simulink model "ASM_Traffic_MultiCore"  (R2026a)
settings: Solver=ode1  StartTime=SIM.tstart.v  StopTime=SIM.tend.v  FixedStep=SIM.StepSize.v
PostLoadFcn:
  | if any(exist('dsrtsu_mdlpostloadfcn', 'file') ~= 0), dsrtsu_mdlpostloadfcn('Execute', bdroot); end
  | try, asm_mdl_postloadfcn(bdroot, 'UpdateModel', 3600); catch, disp(lasterr); end,
InitFcn:
  | , if any(exist('rtifpga_mdlclblib', 'file') ~= 0), rtifpga_mdlclblib('Init', bdroot); end,
  | , if any(exist('dsmpb_private', 'file') ~= 0), dsmpb_private('dsmpb_mdlclblib', 'Init', bdroot); end,
model workspace (MAT data in the model file):
  asmReferencePath = [0 0.01 0.02 0.03 0.04 0.05 0.06 0.07 0.08 0.09 0.1 0.11 ... (350007 elements, 50001x7)]
  roadBounds : Simulink.Parameter (value not decoded)
  safetyAxes : Simulink.Parameter (value not decoded)
undefined symbols (not defined in the file): _to_, a0b2, ASM_BrakeHydraulics_DemoSystems, ASM_VehicleDynamics_DemoSystems, b98103fe8ad365046cd0, BrakeCircuit, controllerConfig, CPT, Crankshaft, DiscIntNeverNeededParam, dsmsi, FinalDriveAssembly, MDL, ModeSignals, mu, Pos_BrakePedal_Maneuver, rad, RefSignals, roadFamilyData, roadFamilyId, s_to_rpm, SIM, SoftECU, Suspension, Tire, Transmission
libraries: ASM_Traffic_lib x135, simulink x98, ASM_Utils_lib x77, ASM_VehicleDynamics_lib x70, ASM_Environment_lib x22, dsmpblib x20, dsmsilib x15, MDLD_Utils_lib x10, ASM_BrakeHydraulics_lib x3, sl_discontinuities x2
(part 43 of 65)

== system ASM_Traffic_MultiCore/Environment/Traffic/PlantModel/FellowMovement/Customize_UserSignals ==
  UserSignals_In : Inport
  UserSignalsFellow_In : Inport  Port=2
  Bus Creator : BusCreator  Inputs=3
  Bus Creator1 : BusCreator  Inputs=213
  Bus Selector : BusSelector  OutputSignals=User1[]
  Bus Selector1 : BusSelector  OutputSignals=User2[],User3[],User4[]
  Bus Selector2 : BusSelector  OutputSignals=User1[],User2[],User3[],User4[],User5[],User6[],User7[],User8[],User9[],User10[]
  Demux{,1..6} (7 alike) : Demux  Outputs=MDL.Traffic.MaxNumFellows.v
  Gain : Gain
  Gain1 : Gain
  Gain2 : Gain
  Memory : UnitDelay  SampleTime=-1
  Mux : Mux  Inputs=10
  Saturation : Saturate  UpperLimit=1  LowerLimit=0
  Select_1 : Selector  InputPortWidth=MDL.Traffic.MaxNumFellows.v*MDL.Traffic.MaxNumFDUserSignals.v  IndexOptions=Index vector (dialog)  Indices=[1:MDL.Traffic.MaxNumFDUserSignals.v:MDL.Traffic.MaxNumFellows.v*MDL.Traffic.MaxNumFDUserSignals.v]  OutputSizes=1
  Select_2 : Selector  InputPortWidth=MDL.Traffic.MaxNumFellows.v*MDL.Traffic.MaxNumFDUserSignals.v  IndexOptions=Index vector (dialog)  Indices=[2:MDL.Traffic.MaxNumFDUserSignals.v:MDL.Traffic.MaxNumFellows.v*MDL.Traffic.MaxNumFDUserSignals.v]  OutputSizes=1
  Select_3 : Selector  InputPortWidth=MDL.Traffic.MaxNumFellows.v*MDL.Traffic.MaxNumFDUserSignals.v  IndexOptions=Index vector (dialog)  Indices=[3:MDL.Traffic.MaxNumFDUserSignals.v:MDL.Traffic.MaxNumFellows.v*MDL.Traffic.MaxNumFDUserSignals.v]  OutputSizes=1
  Select_4 : Selector  InputPortWidth=MDL.Traffic.MaxNumFellows.v*MDL.Traffic.MaxNumFDUserSignals.v  IndexOptions=Index vector (dialog)  Indices=[4:MDL.Traffic.MaxNumFDUserSignals.v:MDL.Traffic.MaxNumFellows.v*MDL.Traffic.MaxNumFDUserSignals.v]  OutputSizes=1
  Select_5 : Selector  InputPortWidth=MDL.Traffic.MaxNumFellows.v*MDL.Traffic.MaxNumFDUserSignals.v  IndexOptions=Index vector (dialog)  Indices=[5:MDL.Traffic.MaxNumFDUserSignals.v:MDL.Traffic.MaxNumFellows.v*MDL.Traffic.MaxNumFDUserSignals.v]  OutputSizes=1
  Select_6 : Selector  InputPortWidth=MDL.Traffic.MaxNumFellows.v*MDL.Traffic.MaxNumFDUserSignals.v  IndexOptions=Index vector (dialog)  Indices=[6:MDL.Traffic.MaxNumFDUserSignals.v:MDL.Traffic.MaxNumFellows.v*MDL.Traffic.MaxNumFDUserSignals.v]  OutputSizes=1
  Select_7 : Selector  InputPortWidth=MDL.Traffic.MaxNumFellows.v*MDL.Traffic.MaxNumFDUserSignals.v  IndexOptions=Index vector (dialog)  Indices=[7:MDL.Traffic.MaxNumFDUserSignals.v:MDL.Traffic.MaxNumFellows.v*MDL.Traffic.MaxNumFDUserSignals.v]  OutputSizes=1
  Select_8 : Selector  InputPortWidth=MDL.Traffic.MaxNumFellows.v*MDL.Traffic.MaxNumFDUserSignals.v  IndexOptions=Index vector (dialog)  Indices=[8:MDL.Traffic.MaxNumFDUserSignals.v:MDL.Traffic.MaxNumFellows.v*MDL.Traffic.MaxNumFDUserSignals.v]  OutputSizes=1
  Sum : Sum  Inputs=|-+  SaturateOnIntegerOverflow=on
  ASMSignalBus : Outport  VectorParamsAs1DForOutWhenUnconnected=off
  Movement_Characteristics[] : Outport  Port=2  VectorParamsAs1DForOutWhenUnconnected=off
  wires:
  Select_2/1 -> Movement_Characteristics[]/1
  Select_1/1 -> Demux/1
  UserSignalsFellow_In/1 -> Select_1/1, Select_2/1, Select_3/1, Select_8/1, Select_7/1, Select_6/1, Select_5/1, Select_4/1
  UserSignals_In/1 -> Bus Selector2/1, Bus Selector1/1, Bus Selector/1  "UserSignals"
  Bus Selector/1 -> Sum/2, Memory/1  "<User1[]>"
  Saturation/1 -> Bus Creator1/1  "ManeuverSegmentEndTrigger[0|1]"
  Bus Creator1/1 -> ASMSignalBus/1  "UserSignals_Customized"
  Sum/1 -> Saturation/1
  Memory/1 -> Sum/1
  Demux/1 -> Bus Creator1/4  "Fellow1_TurnLights"
  Demux/30 -> Bus Creator1/33  "Fellow30_TurnLights"
  Demux/2 -> Bus Creator1/5  "Fellow2_TurnLights"
  Demux/3 -> Bus Creator1/6  "Fellow3_TurnLights"
  Demux/4 -> Bus Creator1/7  "Fellow4_TurnLights"
  Demux/5 -> Bus Creator1/8  "Fellow5_TurnLights"
  Demux/6 -> Bus Creator1/9  "Fellow6_TurnLights"
  Demux/7 -> Bus Creator1/10  "Fellow7_TurnLights"
  Demux/8 -> Bus Creator1/11  "Fellow8_TurnLights"
  Demux/9 -> Bus Creator1/12  "Fellow9_TurnLights"
  Demux/10 -> Bus Creator1/13  "Fellow10_TurnLights"
  Demux/11 -> Bus Creator1/14  "Fellow11_TurnLights"
  Demux/12 -> Bus Creator1/15  "Fellow12_TurnLights"
  Demux/13 -> Bus Creator1/16  "Fellow13_TurnLights"
  Demux/14 -> Bus Creator1/17  "Fellow14_TurnLights"
  Demux/15 -> Bus Creator1/18  "Fellow15_TurnLights"
  Demux/16 -> Bus Creator1/19  "Fellow16_TurnLights"
  Demux/17 -> Bus Creator1/20  "Fellow17_TurnLights"
  Demux/18 -> Bus Creator1/21  "Fellow18_TurnLights"
  Demux/19 -> Bus Creator1/22  "Fellow19_TurnLights"
  Demux/20 -> Bus Creator1/23  "Fellow20_TurnLights"
  Demux/21 -> Bus Creator1/24  "Fellow21_TurnLights"
  Demux/22 -> Bus Creator1/25  "Fellow22_TurnLights"
  Demux/23 -> Bus Creator1/26  "Fellow23_TurnLights"
  Demux/24 -> Bus Creator1/27  "Fellow24_TurnLights"
  Demux/25 -> Bus Creator1/28  "Fellow25_TurnLights"
  Demux/26 -> Bus Creator1/29  "Fellow26_TurnLights"
  Demux/27 -> Bus Creator1/30  "Fellow27_TurnLights"
  Demux/28 -> Bus Creator1/31  "Fellow28_TurnLights"
  Demux/29 -> Bus Creator1/32  "Fellow29_TurnLights"
  Bus Selector2/1 -> Mux/1  "<User1[]>"
  Bus Selector2/2 -> Mux/2  "<User2[]>"
  Bus Selector2/3 -> Mux/3  "<User3[]>"
  Bus Selector2/4 -> Mux/4  "<User4[]>"
  Bus Selector2/5 -> Mux/5  "<User5[]>"
  Mux/1 -> Bus Creator1/3  "UserSignals"
  Demux1/30 -> Bus Creator1/63  "Fellow30_DoorFL"
  Demux1/27 -> Bus Creator1/60  "Fellow27_DoorFL"
  Demux1/25 -> Bus Creator1/58  "Fellow25_DoorFL"
  Demux1/28 -> Bus Creator1/61  "Fellow28_DoorFL"
  Demux1/24 -> Bus Creator1/57  "Fellow24_DoorFL"
  Demux1/29 -> Bus Creator1/62  "Fellow29_DoorFL"
  Demux1/22 -> Bus Creator1/55  "Fellow22_DoorFL"
  Demux1/20 -> Bus Creator1/53  "Fellow20_DoorFL"
  Demux1/21 -> Bus Creator1/54  "Fellow21_DoorFL"
  Demux1/23 -> Bus Creator1/56  "Fellow23_DoorFL"
  Demux1/19 -> Bus Creator1/52  "Fellow19_DoorFL"
  Demux1/18 -> Bus Creator1/51  "Fellow18_DoorFL"
  Demux1/16 -> Bus Creator1/49  "Fellow16_DoorFL"
  Demux1/15 -> Bus Creator1/48  "Fellow15_DoorFL"
  Demux1/12 -> Bus Creator1/45  "Fellow12_DoorFL"
  Demux1/17 -> Bus Creator1/50  "Fellow17_DoorFL"
  Demux1/11 -> Bus Creator1/44  "Fellow11_DoorFL"
  Demux1/9 -> Bus Creator1/42  "Fellow9_DoorFL"
  Demux1/10 -> Bus Creator1/43  "Fellow10_DoorFL"
  Demux1/13 -> Bus Creator1/46  "Fellow13_DoorFL"
  Demux1/3 -> Bus Creator1/36  "Fellow3_DoorFL"
  Select_3/1 -> Demux1/1
  Demux1/7 -> Bus Creator1/40  "Fellow7_DoorFL"
  Demux1/8 -> Bus Creator1/41  "Fellow8_DoorFL"
  Demux1/26 -> Bus Creator1/59  "Fellow26_DoorFL"
  Demux1/6 -> Bus Creator1/39  "Fellow6_DoorFL"
  Demux1/14 -> Bus Creator1/47  "Fellow14_DoorFL"
  Demux1/2 -> Bus Creator1/35  "Fellow2_DoorFL"
  Demux1/5 -> Bus Creator1/38  "Fellow5_DoorFL"
  Demux1/4 -> Bus Creator1/37  "Fellow4_DoorFL"
  Demux1/1 -> Bus Creator1/34  "Fellow1_DoorFL"
  Demux2/30 -> Bus Creator1/93  "Fellow30_DoorFR"
  Demux2/27 -> Bus Creator1/90  "Fellow27_DoorFR"
  Demux2/25 -> Bus Creator1/88  "Fellow25_DoorFR"
  Demux2/28 -> Bus Creator1/91  "Fellow28_DoorFR"
  Demux2/24 -> Bus Creator1/87  "Fellow24_DoorFR"
  Demux2/29 -> Bus Creator1/92  "Fellow29_DoorFR"
  Demux2/22 -> Bus Creator1/85  "Fellow22_DoorFR"
  Demux2/20 -> Bus Creator1/83  "Fellow20_DoorFR"
  Demux2/21 -> Bus Creator1/84  "Fellow21_DoorFR"
  Demux2/23 -> Bus Creator1/86  "Fellow23_DoorFR"
  Demux2/19 -> Bus Creator1/82  "Fellow19_DoorFR"
  Demux2/18 -> Bus Creator1/81  "Fellow18_DoorFR"
  Demux2/16 -> Bus Creator1/79  "Fellow16_DoorFR"
  Demux2/15 -> Bus Creator1/78  "Fellow15_DoorFR"
  Demux2/12 -> Bus Creator1/75  "Fellow12_DoorFR"
  Demux2/17 -> Bus Creator1/80  "Fellow17_DoorFR"
  Demux2/11 -> Bus Creator1/74  "Fellow11_DoorFR"
  Demux2/9 -> Bus Creator1/72  "Fellow9_DoorFR"
  Demux2/10 -> Bus Creator1/73  "Fellow10_DoorFR"
  Demux2/13 -> Bus Creator1/76  "Fellow13_DoorFR"
  Demux2/3 -> Bus Creator1/66  "Fellow3_DoorFR"
  Select_4/1 -> Demux2/1
  Demux2/7 -> Bus Creator1/70  "Fellow7_DoorFR"
  Demux2/8 -> Bus Creator1/71  "Fellow8_DoorFR"
  Demux2/26 -> Bus Creator1/89  "Fellow26_DoorFR"
  Demux2/6 -> Bus Creator1/69  "Fellow6_DoorFR"
  Demux2/14 -> Bus Creator1/77  "Fellow14_DoorFR"
  Demux2/2 -> Bus Creator1/65  "Fellow2_DoorFR"
  Demux2/5 -> Bus Creator1/68  "Fellow5_DoorFR"
  Demux2/4 -> Bus Creator1/67  "Fellow4_DoorFR"
  Demux2/1 -> Bus Creator1/64  "Fellow1_DoorFR"
  Demux3/30 -> Bus Creator1/123  "Fellow30_DoorRL"
  Demux3/27 -> Bus Creator1/120  "Fellow27_DoorRL"
  Demux3/25 -> Bus Creator1/118  "Fellow25_DoorRL"
  Demux3/28 -> Bus Creator1/121  "Fellow28_DoorRL"
  Demux3/24 -> Bus Creator1/117  "Fellow24_DoorRL"
  Demux3/29 -> Bus Creator1/122  "Fellow29_DoorRL"
  Demux3/22 -> Bus Creator1/115  "Fellow22_DoorRL"
  Demux3/20 -> Bus Creator1/113  "Fellow20_DoorRL"
  Demux3/21 -> Bus Creator1/114  "Fellow21_DoorRL"
  Demux3/23 -> Bus Creator1/116  "Fellow23_DoorRL"
  Demux3/19 -> Bus Creator1/112  "Fellow19_DoorRL"
  Demux3/18 -> Bus Creator1/111  "Fellow18_DoorRL"
  Demux3/16 -> Bus Creator1/109  "Fellow16_DoorRL"
  Demux3/15 -> Bus Creator1/108  "Fellow15_DoorRL"
  Demux3/12 -> Bus Creator1/105  "Fellow12_DoorRL"
  Demux3/17 -> Bus Creator1/110  "Fellow17_DoorRL"
  Demux3/11 -> Bus Creator1/104  "Fellow11_DoorRL"
  Demux3/9 -> Bus Creator1/102  "Fellow9_DoorRL"
  Demux3/10 -> Bus Creator1/103  "Fellow10_DoorRL"
  Demux3/13 -> Bus Creator1/106  "Fellow13_DoorRL"
  Demux3/3 -> Bus Creator1/96  "Fellow3_DoorRL"
  Select_5/1 -> Demux3/1
  Demux3/7 -> Bus Creator1/100  "Fellow7_DoorRL"
  Demux3/8 -> Bus Creator1/101  "Fellow8_DoorRL"
  Demux3/26 -> Bus Creator1/119  "Fellow26_DoorRL"
  Demux3/6 -> Bus Creator1/99  "Fellow6_DoorRL"
  Demux3/14 -> Bus Creator1/107  "Fellow14_DoorRL"
  Demux3/2 -> Bus Creator1/95  "Fellow2_DoorRL"
  Demux3/5 -> Bus Creator1/98  "Fellow5_DoorRL"
  Demux3/4 -> Bus Creator1/97  "Fellow4_DoorRL"
  Demux3/1 -> Bus Creator1/94  "Fellow1_DoorRL"
  Demux4/30 -> Bus Creator1/153  "Fellow30_DoorRR"
  Demux4/27 -> Bus Creator1/150  "Fellow27_DoorRR"
  Demux4/25 -> Bus Creator1/148  "Fellow25_DoorRR"
  Demux4/28 -> Bus Creator1/151  "Fellow28_DoorRR"
  Demux4/24 -> Bus Creator1/147  "Fellow24_DoorRR"
  Demux4/29 -> Bus Creator1/152  "Fellow29_DoorRR"
  Demux4/22 -> Bus Creator1/145  "Fellow22_DoorRR"
  Demux4/20 -> Bus Creator1/143  "Fellow20_DoorRR"
  Demux4/21 -> Bus Creator1/144  "Fellow21_DoorRR"
  Demux4/23 -> Bus Creator1/146  "Fellow23_DoorRR"
  Demux4/19 -> Bus Creator1/142  "Fellow19_DoorRR"
  Demux4/18 -> Bus Creator1/141  "Fellow18_DoorRR"
  Demux4/16 -> Bus Creator1/139  "Fellow16_DoorRR"
  Demux4/15 -> Bus Creator1/138  "Fellow15_DoorRR"
  Demux4/12 -> Bus Creator1/135  "Fellow12_DoorRR"
  Demux4/17 -> Bus Creator1/140  "Fellow17_DoorRR"
  Demux4/11 -> Bus Creator1/134  "Fellow11_DoorRR"
  Demux4/9 -> Bus Creator1/132  "Fellow9_DoorRR"
  Demux4/10 -> Bus Creator1/133  "Fellow10_DoorRR"
  Demux4/13 -> Bus Creator1/136  "Fellow13_DoorRR"
  Demux4/3 -> Bus Creator1/126  "Fellow3_DoorRR"
  Select_6/1 -> Demux4/1
  Demux4/7 -> Bus Creator1/130  "Fellow7_DoorRR"
  Demux4/8 -> Bus Creator1/131  "Fellow8_DoorRR"
  Demux4/26 -> Bus Creator1/149  "Fellow26_DoorRR"
  Demux4/6 -> Bus Creator1/129  "Fellow6_DoorRR"
  Demux4/14 -> Bus Creator1/137  "Fellow14_DoorRR"
  Demux4/2 -> Bus Creator1/125  "Fellow2_DoorRR"
  Demux4/5 -> Bus Creator1/128  "Fellow5_DoorRR"
  Demux4/4 -> Bus Creator1/127  "Fellow4_DoorRR"
  Demux4/1 -> Bus Creator1/124  "Fellow1_DoorRR"
  Demux5/30 -> Bus Creator1/183  "Fellow30_Hood"
  Demux5/27 -> Bus Creator1/180  "Fellow27_Hood"
  Demux5/25 -> Bus Creator1/178  "Fellow25_Hood"
  Demux5/28 -> Bus Creator1/181  "Fellow28_Hood"
  Demux5/24 -> Bus Creator1/177  "Fellow24_Hood"
  Demux5/29 -> Bus Creator1/182  "Fellow29_Hood"
  Demux5/22 -> Bus Creator1/175  "Fellow22_Hood"
  Demux5/20 -> Bus Creator1/173  "Fellow20_Hood"
  Demux5/21 -> Bus Creator1/174  "Fellow21_Hood"
  Demux5/23 -> Bus Creator1/176  "Fellow23_Hood"
  Demux5/19 -> Bus Creator1/172  "Fellow19_Hood"
  Demux5/18 -> Bus Creator1/171  "Fellow18_Hood"
  Demux5/16 -> Bus Creator1/169  "Fellow16_Hood"
  Demux5/15 -> Bus Creator1/168  "Fellow15_Hood"
  Demux5/12 -> Bus Creator1/165  "Fellow12_Hood"
  Demux5/17 -> Bus Creator1/170  "Fellow17_Hood"
  Demux5/11 -> Bus Creator1/164  "Fellow11_Hood"
  Demux5/9 -> Bus Creator1/162  "Fellow9_Hood"
  Demux5/10 -> Bus Creator1/163  "Fellow10_Hood"
  Demux5/13 -> Bus Creator1/166  "Fellow13_Hood"
  Demux5/3 -> Bus Creator1/156  "Fellow3_Hood"
  Select_7/1 -> Demux5/1
  Demux5/7 -> Bus Creator1/160  "Fellow7_Hood"
  Demux5/8 -> Bus Creator1/161  "Fellow8_Hood"
  Demux5/26 -> Bus Creator1/179  "Fellow26_Hood"
  Demux5/6 -> Bus Creator1/159  "Fellow6_Hood"
  Demux5/14 -> Bus Creator1/167  "Fellow14_Hood"
  Demux5/2 -> Bus Creator1/155  "Fellow2_Hood"
  Demux5/5 -> Bus Creator1/158  "Fellow5_Hood"
  Demux5/4 -> Bus Creator1/157  "Fellow4_Hood"
  Demux5/1 -> Bus Creator1/154  "Fellow1_Hood"
  Demux6/30 -> Bus Creator1/213  "Fellow30_Trunk"
  Demux6/27 -> Bus Creator1/210  "Fellow27_Trunk"
  Demux6/25 -> Bus Creator1/208  "Fellow25_Trunk"
  Demux6/28 -> Bus Creator1/211  "Fellow28_Trunk"
  Demux6/24 -> Bus Creator1/207  "Fellow24_Trunk"
  Demux6/29 -> Bus Creator1/212  "Fellow29_Trunk"
  Demux6/22 -> Bus Creator1/205  "Fellow22_Trunk"
  Demux6/20 -> Bus Creator1/203  "Fellow20_Trunk"
  Demux6/21 -> Bus Creator1/204  "Fellow21_Trunk"
  Demux6/23 -> Bus Creator1/206  "Fellow23_Trunk"
  Demux6/19 -> Bus Creator1/202  "Fellow19_Trunk"
  Demux6/18 -> Bus Creator1/201  "Fellow18_Trunk"
  Demux6/16 -> Bus Creator1/199  "Fellow16_Trunk"
  Demux6/15 -> Bus Creator1/198  "Fellow15_Trunk"
  Demux6/12 -> Bus Creator1/195  "Fellow12_Trunk"
  Demux6/17 -> Bus Creator1/200  "Fellow17_Trunk"
  Demux6/11 -> Bus Creator1/194  "Fellow11_Trunk"
  Demux6/9 -> Bus Creator1/192  "Fellow9_Trunk"
  Demux6/10 -> Bus Creator1/193  "Fellow10_Trunk"
  Demux6/13 -> Bus Creator1/196  "Fellow13_Trunk"
  Demux6/3 -> Bus Creator1/186  "Fellow3_Trunk"
  Select_8/1 -> Demux6/1
  Demux6/7 -> Bus Creator1/190  "Fellow7_Trunk"
  Demux6/8 -> Bus Creator1/191  "Fellow8_Trunk"
  Demux6/26 -> Bus Creator1/209  "Fellow26_Trunk"
  Demux6/6 -> Bus Creator1/189  "Fellow6_Trunk"
  Demux6/14 -> Bus Creator1/197  "Fellow14_Trunk"
  Demux6/2 -> Bus Creator1/185  "Fellow2_Trunk"
  Demux6/5 -> Bus Creator1/188  "Fellow5_Trunk"
  Demux6/4 -> Bus Creator1/187  "Fellow4_Trunk"
  Demux6/1 -> Bus Creator1/184  "Fellow1_Trunk"
  Bus Selector2/6 -> Mux/6  "<User6[]>"
  Bus Selector2/7 -> Mux/7  "<User7[]>"
  Bus Selector2/8 -> Mux/8  "<User8[]>"
  Bus Selector1/1 -> Gain/1  "<User2[]>"
  Bus Creator/1 -> Bus Creator1/2  "DriverMonitoring"
  Bus Selector1/2 -> Gain1/1  "<User3[]>"
  Bus Selector1/3 -> Gain2/1  "<User4[]>"
  Bus Selector2/10 -> Mux/10  "<User10[]>"
  Bus Selector2/9 -> Mux/9  "<User9[]>"
  Gain/1 -> Bus Creator/1  "DriverGazeLocation[]"
  Gain1/1 -> Bus Creator/2  "DriverAnimation[]"
  Gain2/1 -> Bus Creator/3  "DriverLizardOwlRatio[]"

== system ASM_Traffic_MultiCore/Environment/Traffic/PlantModel/FellowMovement/External_Route ==
  Const_RouteDirection_Fellows_External[] : Constant  Value=zeros(1,MDL.Traffic.MaxNumFellows.v)
  Const_RouteId_Fellows_External[] : Constant  Value=zeros(1,MDL.Traffic.MaxNumFellows.v)
  RouteId_External[] : Outport  VectorParamsAs1DForOutWhenUnconnected=off
  RouteDirection_External[1|-1] : Outport  Port=2  VectorParamsAs1DForOutWhenUnconnected=off
  wires:
  Const_RouteDirection_Fellows_External[]/1 -> RouteDirection_External[1|-1]/1
  Const_RouteId_Fellows_External[]/1 -> RouteId_External[]/1

== system ASM_Traffic_MultiCore/Environment/Traffic/PlantModel/FellowMovement/External_Signals ==
  Const_LaneIdx_Fellows_External[] : Constant  Value=zeros(1,MDL.Traffic.MaxNumFellows.v)
  Const_d_Fellows_External[m] : Constant  Value=zeros(1,MDL.Traffic.MaxNumFellows.v)
  Const_s_Fellows_External[m] : Constant  Value=zeros(1,MDL.Traffic.MaxNumFellows.v)
  Const_tgap_Fellows_External[s] : Constant  Value=zeros(1,MDL.Traffic.MaxNumFellows.v)
  Const_v_Fellows_External[km|h] : Constant  Value=zeros(1,MDL.Traffic.MaxNumFellows.v)
  s_Fellows_External[m] : Outport  VectorParamsAs1DForOutWhenUnconnected=off
  v_Fellows_External[km|h] : Outport  Port=2  VectorParamsAs1DForOutWhenUnconnected=off
  d_Fellows_External[m] : Outport  Port=3  VectorParamsAs1DForOutWhenUnconnected=off
  tgap_Fellows_External[s] : Outport  Port=4  VectorParamsAs1DForOutWhenUnconnected=off
  LaneIdx_Fellows_External[] : Outport  Port=5  VectorParamsAs1DForOutWhenUnconnected=off
  wires:
  Const_LaneIdx_Fellows_External[]/1 -> LaneIdx_Fellows_External[]/1
  Const_tgap_Fellows_External[s]/1 -> tgap_Fellows_External[s]/1
  Const_v_Fellows_External[km|h]/1 -> v_Fellows_External[km|h]/1
  Const_d_Fellows_External[m]/1 -> d_Fellows_External[m]/1
  Const_s_Fellows_External[m]/1 -> s_Fellows_External[m]/1

== system ASM_Traffic_MultiCore/Environment/Traffic/PlantModel/FellowMovement/LabelUserSignals ==
  UserSignals_In : Inport
  Bus Creator : BusCreator  Inputs=10
  UserSignals_ : Subsystem
  UserSignals : Outport  VectorParamsAs1DForOutWhenUnconnected=off
  wires:
  UserSignals_In/1 -> UserSignals_/1(UserSignals)
  Bus Creator/1 -> UserSignals/1  "UserSignals"
  UserSignals_/1(User1[]) -> Bus Creator/1  "User1[]"
  UserSignals_/5(User5[]) -> Bus Creator/5  "User5[]"
  UserSignals_/6(User6[]) -> Bus Creator/6  "User6[]"
  UserSignals_/7(User7[]) -> Bus Creator/7  "User7[]"
  UserSignals_/8(User8[]) -> Bus Creator/8  "User8[]"
  UserSignals_/9(User9[]) -> Bus Creator/9  "User9[]"
  UserSignals_/10(User10[]) -> Bus Creator/10  "User10[]"
  UserSignals_/2(User2[]) -> Bus Creator/2  "User2[]"
  UserSignals_/3(User3[]) -> Bus Creator/3  "User3[]"
  UserSignals_/4(User4[]) -> Bus Creator/4  "User4[]"

== system ASM_Traffic_MultiCore/Environment/Traffic/PlantModel/FellowMovement/Maneuver_Status_Handling ==
  ManeuverState[] : Inport
  Constant1 : Constant  Value=3
  Constant2 : Constant  Value=2
  Constant3 : Constant  Value=5
  Constant4 : Constant  Value=5
  Constant5 : Constant
  Constant6 : Constant  Value=0
  Constant7 : Constant  Value=2
  Constant8 : Constant  Value=0
  Logical Operator : Logic  AllPortsSameDT=off
  Logical Operator1 : Logic  AllPortsSameDT=off
  Memory : UnitDelay  SampleTime=-1
  Relational Operator : RelationalOperator  Operator===
  Relational Operator1 : RelationalOperator  Operator===
  Relational Operator2 : RelationalOperator  Operator===
  Relational Operator3 : RelationalOperator  Operator=~=
  Start : MultiPortSwitch  DataPortOrder=Zero-based contiguous  Inputs=2  zeroidx=on  InputSameDT=off
  "Stop " : MultiPortSwitch  DataPortOrder=Zero-based contiguous  Inputs=2  zeroidx=on  InputSameDT=off
  Sum1 : Sum  Inputs=|++  SaturateOnIntegerOverflow=on
  Traffic_Ctrl : Outport  VectorParamsAs1DForOutWhenUnconnected=off
  wires:
  Sum1/1 -> Traffic_Ctrl/1  "handling"
  ManeuverState[]/1 -> Relational Operator2/1, Relational Operator/1, Memory/1  "status"
  "Stop "/1 -> Sum1/2  "stop"
  Constant7/1 -> "Stop "/3
  Constant8/1 -> "Stop "/2
  Logical Operator1/1 -> "Stop "/1  "stop"
  Start/1 -> Sum1/1  "start"
  Constant5/1 -> Start/3
  Constant6/1 -> Start/2
  Logical Operator/1 -> Start/1
  Relational Operator3/1 -> Logical Operator1/2
  Relational Operator2/1 -> Logical Operator1/1
  Constant4/1 -> Relational Operator3/2
  Constant3/1 -> Relational Operator2/2
  Relational Operator1/1 -> Logical Operator/2
  Relational Operator/1 -> Logical Operator/1
  Constant2/1 -> Relational Operator1/2
  Constant1/1 -> Relational Operator/2
  Memory/1 -> Relational Operator3/1, Relational Operator1/1

== system ASM_Traffic_MultiCore/Environment/Traffic/PlantModel/FellowMovement/ObjectParameters_Modified ==
  ObjectParameters_Signals_In : Inport
  s_Fellows_Scheduler[m] : Inport  Port=2
  Movement_Characteristics[] : Inport  Port=3
  Bus Creator : BusCreator  Inputs=4
  Bus Creator1 : BusCreator  Inputs=1
  Bus Selector : BusSelector  OutputSignals=FellowParameters.Length_Fellows[m],FellowParameters.Wheel_Radius_Fellows[m]
  MATLAB Function : MATLAB Function  TreatAsAtomicUnit=on
  Yaw_Angle_Correction_Handling : Subsystem
  use_yaw_road[0|1] : Outport  VectorParamsAs1DForOutWhenUnconnected=off
  ObjectParameters_Signals : Outport  Port=2  VectorParamsAs1DForOutWhenUnconnected=off
  wires:
  Bus Creator1/1 -> ObjectParameters_Signals/1
  Bus Creator/1 -> Bus Creator1/1  "FellowParameters"
  MATLAB Function/1(hitch_dist) -> Bus Creator/4  "Hitch_Dist[m]"
  Movement_Characteristics[]/1 -> Yaw_Angle_Correction_Handling/1(Movement_Characteristics[]), Bus Creator/3  "Movement_Characteristics[]"
  Bus Selector/2 -> Bus Creator/2  "<Wheel_Radius_Fellows[m]>"
  Bus Selector/1 -> Bus Creator/1  "<Length_Fellows[m]>"
  s_Fellows_Scheduler[m]/1 -> MATLAB Function/1(s_fellow_m)
  ObjectParameters_Signals_In/1 -> Bus Selector/1
  Yaw_Angle_Correction_Handling/1(use_yaw_road[0|1]) -> use_yaw_road[0|1]/1

== system ASM_Traffic_MultiCore/Environment/Traffic/PlantModel/FellowMovement/Objects_DataStreams ==
  Objects_DataStreams_In[] : Inport
  Bus Selector : BusSelector  OutputSignals=DataStream_1[].DataStream_1[],DataStream_2[].DataStream_2[],DataStream_3[].DataStream_3[],DataStream_4[].DataStream_4[],DataStream_5[].DataStream_5[],DataStream_6[].DataStream_6[],DataStream_7[].DataStream_7[],DataStream_8[].DataStream_8[]
  Mux : Mux  Inputs=8
  Objects_DataStreams[] : Outport  VectorParamsAs1DForOutWhenUnconnected=off
  wires:
  Objects_DataStreams_In[]/1 -> Bus Selector/1
  Bus Selector/8 -> Mux/8  "<DataStream_8[]>"
  Bus Selector/7 -> Mux/7  "<DataStream_7[]>"
  Bus Selector/6 -> Mux/6  "<DataStream_6[]>"
  Bus Selector/5 -> Mux/5  "<DataStream_5[]>"
  Bus Selector/4 -> Mux/4  "<DataStream_4[]>"
  Bus Selector/3 -> Mux/3  "<DataStream_3[]>"
  Bus Selector/2 -> Mux/2  "<DataStream_2[]>"
  Bus Selector/1 -> Mux/1  "<DataStream_1[]>"
  Mux/1 -> Objects_DataStreams[]/1  "Objects_DataStreams[]"

== system ASM_Traffic_MultiCore/Environment/Traffic/PlantModel/FellowMovement/SegmentEnd_External ==
  Const_SegmentEnd_External1[0|1] : Constant  Value=0
  Const_SegmentEnd_External2[0|1] : Constant  Value=0
  Const_SegmentEnd_External3[0|1] : Constant  Value=0
  Mux3 : Mux  Inputs=3
  SegmentEnd_External[0|1] : Outport  VectorParamsAs1DForOutWhenUnconnected=off
  wires:
  Mux3/1 -> SegmentEnd_External[0|1]/1
  Const_SegmentEnd_External1[0|1]/1 -> Mux3/1
  Const_SegmentEnd_External2[0|1]/1 -> Mux3/2
  Const_SegmentEnd_External3[0|1]/1 -> Mux3/3

== system ASM_Traffic_MultiCore/Environment/Traffic/PlantModel/FellowMovement/Sw_SpeedLimit_Enable ==
  SpeedLimit_In : Inport
  Multiport Switch : MultiPortSwitch  DataPortOrder=Zero-based contiguous  Inputs=2  DiagnosticForDefault=Warning  zeroidx=on  SaturateOnIntegerOverflow=off  InputSameDT=off
  SpeedLimit_Off[km|h] : Constant  Value=1000.0
  SpeedLimit_RateLimiter : Subsystem
  Sw_SpeedLimit_Enable[0Off|1On] : Constant  Value=[ones(1,MDL.Traffic.MaxNumFellows.v)]  OutDataTypeStr=uint8
  SpeedLimit_Out : Outport  VectorParamsAs1DForOutWhenUnconnected=off
  wires:
  SpeedLimit_In/1 -> SpeedLimit_RateLimiter/1(In)
  SpeedLimit_RateLimiter/1(Out) -> Multiport Switch/3
  SpeedLimit_Off[km|h]/1 -> Multiport Switch/2
  Multiport Switch/1 -> SpeedLimit_Out/1
  Sw_SpeedLimit_Enable[0Off|1On]/1 -> Multiport Switch/1

== system ASM_Traffic_MultiCore/Environment/Traffic/PlantModel/Merge_Signals_toEnvironment/avoid_incomplete_trace2source ==
  In1 : Inport
  Bus Creator : BusCreator  Inputs=6
  Bus Selector : BusSelector  OutputSignals=Quadrant_Def_Mode[1Internal|2External],Quadrant_Dim_x[m],Quadrant_Dim_y[m],Interface_Mode[0Off|1ObjOnly|2ObjAndLanes],Interface_Init[0Off|1On],Interface_Init_Ready[0Off|1On]
  avoid_incomplete_trace2source : Subsystem
  avoid_incomplete_trace2source1 : Subsystem
  avoid_incomplete_trace2source2 : Subsystem
  avoid_incomplete_trace2source3 : Subsystem
  avoid_incomplete_trace2source4 : Subsystem
  avoid_incomplete_trace2source5 : Subsystem
  Out1 : Outport
  wires:
  avoid_incomplete_trace2source5/1(Out1) -> Bus Creator/6  "Interface_Init_Ready[0Off|1On]"
  avoid_incomplete_trace2source4/1(Out1) -> Bus Creator/5  "Interface_Init[0Off|1On]"
  avoid_incomplete_trace2source3/1(Out1) -> Bus Creator/4  "Interface_Mode[0Off|1ObjOnly|2ObjAndLanes]"
  avoid_incomplete_trace2source2/1(Out1) -> Bus Creator/3  "Quadrant_Dim_y[m]"
  avoid_incomplete_trace2source1/1(Out1) -> Bus Creator/2  "Quadrant_Dim_x[m]"
  avoid_incomplete_trace2source/1(Out1) -> Bus Creator/1  "Quadrant_Def_Mode[1Internal|2External]"
  Bus Creator/1 -> Out1/1
  Bus Selector/2 -> avoid_incomplete_trace2source1/1(In1)  "<Quadrant_Dim_x[m]>"
  Bus Selector/3 -> avoid_incomplete_trace2source2/1(In1)  "<Quadrant_Dim_y[m]>"
  Bus Selector/4 -> avoid_incomplete_trace2source3/1(In1)  "<Interface_Mode[0Off|1ObjOnly|2ObjAndLanes]>"
  Bus Selector/5 -> avoid_incomplete_trace2source4/1(In1)  "<Interface_Init[0Off|1On]>"
  Bus Selector/6 -> avoid_incomplete_trace2source5/1(In1)  "<Interface_Init_Ready[0Off|1On]>"
  Bus Selector/1 -> avoid_incomplete_trace2source/1(In1)  "<Quadrant_Def_Mode[1Internal|2External]>"
  In1/1 -> Bus Selector/1

== system ASM_Traffic_MultiCore/Environment/Traffic/PlantModel/ObjectParameters/ASMSignalCollector ==
  Bus Creator1 : BusCreator  Inputs=3
  ObjectParameter_Signals : Outport  VectorParamsAs1DForOutWhenUnconnected=off
  wires:
  [ASMBUS_Environment_Traffic_DiscreteObjects] -> Bus Creator1/3  "DiscreteObjects"
  Bus Creator1/1 -> ObjectParameter_Signals/1  "ObjectParameters"
  [ASMBUS_Environment_Traffic_FellowParameters] -> Bus Creator1/1  "FellowParameters"
  [ASMBUS_Environment_Traffic_TrafficObjects] -> Bus Creator1/2  "TrafficObjects"

== system ASM_Traffic_MultiCore/Environment/Traffic/PlantModel/ObjectParameters/TrafficObject_Reload_Trigger ==
  RoadState[] : Inport
  RoadControl[] : Inport  Port=2
  Constant1 : Constant  Value=3
  Constant2 : Constant  Value=2
  Constant3 : Constant
  Constant5 : Constant
  Constant6 : Constant  Value=0
  Logical Operator : Logic  Inputs=3  AllPortsSameDT=off
  Memory : UnitDelay  SampleTime=-1
  Relational Operator : RelationalOperator  Operator===
  Relational Operator1 : RelationalOperator  Operator===
  Relational Operator2 : RelationalOperator  Operator===
  Start : MultiPortSwitch  DataPortOrder=Zero-based contiguous  Inputs=2  zeroidx=on  InputSameDT=off
  Ctrl : Outport  VectorParamsAs1DForOutWhenUnconnected=off
  wires:
  Relational Operator2/1 -> Logical Operator/3
  Constant3/1 -> Relational Operator2/2
  RoadControl[]/1 -> Relational Operator2/1
  Memory/1 -> Relational Operator1/1
  Constant1/1 -> Relational Operator/2
  Constant2/1 -> Relational Operator1/2
  Relational Operator/1 -> Logical Operator/1
  Relational Operator1/1 -> Logical Operator/2
  Logical Operator/1 -> Start/1
  Constant6/1 -> Start/2
  Constant5/1 -> Start/3
  Start/1 -> Ctrl/1  "start"
  RoadState[]/1 -> Relational Operator/1, Memory/1  "status"

== system ASM_Traffic_MultiCore/Environment/Traffic/PlantModel/V2X/ASMSignalCollector ==
  Bus Creator1 : BusCreator  Inputs=1
  V2X_Signals : Outport  VectorParamsAs1DForOutWhenUnconnected=off
  wires:
  Bus Creator1/1 -> V2X_Signals/1  "V2X"
  [ASMBUS_Traffic_V2X_TrafficLightController] -> Bus Creator1/1

== system ASM_Traffic_MultiCore/Environment/Traffic/UserInterface/DISP_Plant/Fellow_Movement ==
  TrafficBus : Inport
  CurrentSegment[] : Subsystem
      mask Display: disp('')
  CurrentSegment[]1 : Subsystem
      mask Display: disp('')
  CurrentSegment[]2 : Subsystem
      mask Display: disp('')
  CurrentSequence[] : Subsystem
      mask Display: disp('')
  CurrentSequence[]1 : Subsystem
      mask Display: disp('')
  CurrentSequence[]2 : Subsystem
      mask Display: disp('')
  Fellow_Movement_1 : Scope  NumInputPorts=7
      settings: TimeSpan=5  ActiveDisplayYMinimum=-1.25  ActiveDisplayYMaximum=1.25  DataLoggingMaxPoints=20000  DataLoggingDecimation=10  DataLoggingVariableName=ScopeData21
  Fellow_Movement_2 : Scope  NumInputPorts=7
      settings: TimeSpan=5  ActiveDisplayYMinimum=0.95  ActiveDisplayYMaximum=1.05  DataLoggingMaxPoints=20000  DataLoggingDecimation=10  DataLoggingVariableName=ScopeData22
  Fellow_Movement_3 : Scope  NumInputPorts=7
      settings: TimeSpan=5  ActiveDisplayYMinimum=0.95  ActiveDisplayYMaximum=1.05  DataLoggingMaxPoints=20000  DataLoggingDecimation=10  DataLoggingVariableName=ScopeData23
  FlagFellowUsed[0|1] : Subsystem
      mask Display: disp('')
  FlagFellowUsed[0|1]1 : Subsystem
      mask Display: disp('')
  FlagFellowUsed[0|1]2 : Subsystem
      mask Display: disp('')
  GetFellowDataByIndex_1 : Subsystem
  GetFellowDataByIndex_2 : Subsystem
  GetFellowDataByIndex_3 : Subsystem
  SelectFellowDataByIndex_1 : Constant
  SelectFellowDataByIndex_2 : Constant  Value=2
  SelectFellowDataByIndex_3 : Constant  Value=3
  d_Total_Fellow[m] : Subsystem
      mask Display: disp('')
  d_Total_Fellow[m]1 : Subsystem
      mask Display: disp('')
  d_Total_Fellow[m]2 : Subsystem
      mask Display: disp('')
  s_Fellow[m] : Subsystem
      mask Display: disp('')
  s_Fellow[m]1 : Subsystem
      mask Display: disp('')
  s_Fellow[m]2 : Subsystem
      mask Display: disp('')
  t_local[s] : Subsystem
      mask Display: disp('')
  t_local[s]1 : Subsystem
      mask Display: disp('')
  t_local[s]2 : Subsystem
      mask Display: disp('')
  v_Fellow[km|h] : Subsystem
      mask Display: disp('')
  v_Fellow[km|h]1 : Subsystem
      mask Display: disp('')
  v_Fellow[km|h]2 : Subsystem
      mask Display: disp('')
  wires:
  GetFellowDataByIndex_3/7(v_Fellow[km|h]) -> v_Fellow[km|h]2/1(In1)
  GetFellowDataByIndex_3/6(d_Total_Fellow[m]) -> d_Total_Fellow[m]2/1(In1)
  GetFellowDataByIndex_3/5(s_Fellow[m]) -> s_Fellow[m]2/1(In1)
  GetFellowDataByIndex_3/4(FlagFellowUsed[0|1]) -> FlagFellowUsed[0|1]2/1(In1)
  GetFellowDataByIndex_3/3(t_local[s]) -> t_local[s]2/1(In1)
  GetFellowDataByIndex_3/2(CurrentSegment[]) -> CurrentSegment[]2/1(In1)
  GetFellowDataByIndex_3/1(CurrentSequence[]) -> CurrentSequence[]2/1(In1)
  v_Fellow[km|h]2/1(Out1) -> Fellow_Movement_3/7  "v_Fellow[km|h]2"
  d_Total_Fellow[m]2/1(Out1) -> Fellow_Movement_3/6  "d_Total_Fellow[m]2"
  s_Fellow[m]2/1(Out1) -> Fellow_Movement_3/5  "s_Fellow[m]2"
  FlagFellowUsed[0|1]2/1(Out1) -> Fellow_Movement_3/4  "FlagFellowUsed[0|1]2"
  t_local[s]2/1(Out1) -> Fellow_Movement_3/3  "t_local[s]2"
  CurrentSegment[]2/1(Out1) -> Fellow_Movement_3/2  "CurrentSegment[]2"
  CurrentSequence[]2/1(Out1) -> Fellow_Movement_3/1  "CurrentSequence[]2"
  SelectFellowDataByIndex_3/1 -> GetFellowDataByIndex_3/1(SelectFellowDataByIndex)
  GetFellowDataByIndex_2/7(v_Fellow[km|h]) -> v_Fellow[km|h]1/1(In1)
  GetFellowDataByIndex_2/6(d_Total_Fellow[m]) -> d_Total_Fellow[m]1/1(In1)
  GetFellowDataByIndex_2/5(s_Fellow[m]) -> s_Fellow[m]1/1(In1)
  GetFellowDataByIndex_2/4(FlagFellowUsed[0|1]) -> FlagFellowUsed[0|1]1/1(In1)
  GetFellowDataByIndex_2/3(t_local[s]) -> t_local[s]1/1(In1)
  GetFellowDataByIndex_2/2(CurrentSegment[]) -> CurrentSegment[]1/1(In1)
  GetFellowDataByIndex_2/1(CurrentSequence[]) -> CurrentSequence[]1/1(In1)
  v_Fellow[km|h]1/1(Out1) -> Fellow_Movement_2/7  "v_Fellow[km|h]1"
  d_Total_Fellow[m]1/1(Out1) -> Fellow_Movement_2/6  "d_Total_Fellow[m]1"
  s_Fellow[m]1/1(Out1) -> Fellow_Movement_2/5  "s_Fellow[m]1"
  FlagFellowUsed[0|1]1/1(Out1) -> Fellow_Movement_2/4  "FlagFellowUsed[0|1]1"
  t_local[s]1/1(Out1) -> Fellow_Movement_2/3  "t_local[s]1"
  CurrentSegment[]1/1(Out1) -> Fellow_Movement_2/2  "CurrentSegment[]1"
  CurrentSequence[]1/1(Out1) -> Fellow_Movement_2/1  "CurrentSequence[]1"
  SelectFellowDataByIndex_2/1 -> GetFellowDataByIndex_2/1(SelectFellowDataByIndex)
  GetFellowDataByIndex_1/7(v_Fellow[km|h]) -> v_Fellow[km|h]/1(In1)
  GetFellowDataByIndex_1/6(d_Total_Fellow[m]) -> d_Total_Fellow[m]/1(In1)
  GetFellowDataByIndex_1/5(s_Fellow[m]) -> s_Fellow[m]/1(In1)
  GetFellowDataByIndex_1/4(FlagFellowUsed[0|1]) -> FlagFellowUsed[0|1]/1(In1)
  GetFellowDataByIndex_1/3(t_local[s]) -> t_local[s]/1(In1)
  GetFellowDataByIndex_1/2(CurrentSegment[]) -> CurrentSegment[]/1(In1)
  GetFellowDataByIndex_1/1(CurrentSequence[]) -> CurrentSequence[]/1(In1)
  v_Fellow[km|h]/1(Out1) -> Fellow_Movement_1/7  "v_Fellow[km|h]"
  d_Total_Fellow[m]/1(Out1) -> Fellow_Movement_1/6  "d_Total_Fellow[m]"
  s_Fellow[m]/1(Out1) -> Fellow_Movement_1/5  "s_Fellow[m]"
  FlagFellowUsed[0|1]/1(Out1) -> Fellow_Movement_1/4  "FlagFellowUsed[0|1]"
  t_local[s]/1(Out1) -> Fellow_Movement_1/3  "t_local[s]"
  CurrentSegment[]/1(Out1) -> Fellow_Movement_1/2  "CurrentSegment[]"
  CurrentSequence[]/1(Out1) -> Fellow_Movement_1/1  "CurrentSequence[]"
  SelectFellowDataByIndex_1/1 -> GetFellowDataByIndex_1/1(SelectFellowDataByIndex)
  TrafficBus/1 -> GetFellowDataByIndex_1/2(TrafficBus), GetFellowDataByIndex_2/2(TrafficBus), GetFellowDataByIndex_3/2(TrafficBus)

== system ASM_Traffic_MultiCore/Environment/Traffic/UserInterface/DISP_Plant/TrafficState[] ==
  In1 : Inport
  Out1 : Outport  VectorParamsAs1DForOutWhenUnconnected=off
  wires:
  In1/1 -> Out1/1

== system ASM_Traffic_MultiCore/Environment/Traffic/UserInterface/PAR_Plant/Fellow_Doors ==
  Bus Creator2 : BusCreator  Inputs=30
  Fellow10_Doors : Subsystem
  Fellow11_Doors : Subsystem
  Fellow12_Doors : Subsystem
  Fellow13_Doors : Subsystem
  Fellow14_Doors : Subsystem
  Fellow15_Doors : Subsystem
  Fellow16_Doors : Subsystem
  Fellow17_Doors : Subsystem
  Fellow18_Doors : Subsystem
  Fellow19_Doors : Subsystem
  Fellow1_Doors : Subsystem
  Fellow20_Doors : Subsystem
  Fellow21_Doors : Subsystem
  Fellow22_Doors : Subsystem
  Fellow23_Doors : Subsystem
  Fellow24_Doors : Subsystem
  Fellow25_Doors : Subsystem
  Fellow26_Doors : Subsystem
  Fellow27_Doors : Subsystem
  Fellow28_Doors : Subsystem
  Fellow29_Doors : Subsystem
  Fellow2_Doors : Subsystem
  Fellow30_Doors : Subsystem
  Fellow3_Doors : Subsystem
  Fellow4_Doors : Subsystem
  Fellow5_Doors : Subsystem
  Fellow6_Doors : Subsystem
  Fellow7_Doors : Subsystem
  Fellow8_Doors : Subsystem
  Fellow9_Doors : Subsystem
  Out1 : Outport  VectorParamsAs1DForOutWhenUnconnected=off
  wires:
  Bus Creator2/1 -> Out1/1  "FellowVehicleDoors"
  Fellow1_Doors/1(Out1) -> Bus Creator2/1  "Fellow1_Doors"
  Fellow2_Doors/1(Out1) -> Bus Creator2/2  "Fellow2_Doors"
  Fellow4_Doors/1(Out1) -> Bus Creator2/4  "Fellow4_Doors"
  Fellow3_Doors/1(Out1) -> Bus Creator2/3  "Fellow3_Doors"
  Fellow6_Doors/1(Out1) -> Bus Creator2/6  "Fellow6_Doors"
  Fellow5_Doors/1(Out1) -> Bus Creator2/5  "Fellow5_Doors"
  Fellow8_Doors/1(Out1) -> Bus Creator2/8  "Fellow8_Doors"
  Fellow7_Doors/1(Out1) -> Bus Creator2/7  "Fellow7_Doors"
  Fellow14_Doors/1(Out1) -> Bus Creator2/14  "Fellow14_Doors"
  Fellow10_Doors/1(Out1) -> Bus Creator2/10  "Fellow10_Doors"
  Fellow9_Doors/1(Out1) -> Bus Creator2/9  "Fellow9_Doors"
  Fellow12_Doors/1(Out1) -> Bus Creator2/12  "Fellow12_Doors"
  Fellow16_Doors/1(Out1) -> Bus Creator2/16  "Fellow16_Doors"
  Fellow11_Doors/1(Out1) -> Bus Creator2/11  "Fellow11_Doors"
  Fellow15_Doors/1(Out1) -> Bus Creator2/15  "Fellow15_Doors"
  Fellow13_Doors/1(Out1) -> Bus Creator2/13  "Fellow13_Doors"
  Fellow22_Doors/1(Out1) -> Bus Creator2/22  "Fellow22_Doors"
  Fellow18_Doors/1(Out1) -> Bus Creator2/18  "Fellow18_Doors"
  Fellow28_Doors/1(Out1) -> Bus Creator2/28  "Fellow28_Doors"
  Fellow30_Doors/1(Out1) -> Bus Creator2/30  "Fellow30_Doors"
  Fellow26_Doors/1(Out1) -> Bus Creator2/26  "Fellow26_Doors"
  Fellow27_Doors/1(Out1) -> Bus Creator2/27  "Fellow27_Doors"
  Fellow29_Doors/1(Out1) -> Bus Creator2/29  "Fellow29_Doors"
  Fellow17_Doors/1(Out1) -> Bus Creator2/17  "Fellow17_Doors"
  Fellow20_Doors/1(Out1) -> Bus Creator2/20  "Fellow20_Doors"
  Fellow19_Doors/1(Out1) -> Bus Creator2/19  "Fellow19_Doors"
  Fellow24_Doors/1(Out1) -> Bus Creator2/24  "Fellow24_Doors"
  Fellow23_Doors/1(Out1) -> Bus Creator2/23  "Fellow23_Doors"
  Fellow25_Doors/1(Out1) -> Bus Creator2/25  "Fellow25_Doors"
  Fellow21_Doors/1(Out1) -> Bus Creator2/21  "Fellow21_Doors"

== system ASM_Traffic_MultiCore/Environment/Traffic/UserInterface/PAR_Plant/Fellow_VehicleLights ==
  Bus Creator2 : BusCreator  Inputs=30
  Fellow10_VehicleLights : Subsystem
  Fellow11_VehicleLights : Subsystem
  Fellow12_VehicleLights : Subsystem
  Fellow13_VehicleLights : Subsystem
  Fellow14_VehicleLights : Subsystem
  Fellow15_VehicleLights : Subsystem
  Fellow16_VehicleLights : Subsystem
  Fellow17_VehicleLights : Subsystem
  Fellow18_VehicleLights : Subsystem
  Fellow19_VehicleLights : Subsystem
  Fellow1_VehicleLights : Subsystem
  Fellow20_VehicleLights : Subsystem
  Fellow21_VehicleLights : Subsystem
  Fellow22_VehicleLights : Subsystem
  Fellow23_VehicleLights : Subsystem
  Fellow24_VehicleLights : Subsystem
  Fellow25_VehicleLights : Subsystem
  Fellow26_VehicleLights : Subsystem
  Fellow27_VehicleLights : Subsystem
  Fellow28_VehicleLights : Subsystem
  Fellow29_VehicleLights : Subsystem
  Fellow2_VehicleLights : Subsystem
  Fellow30_VehicleLights : Subsystem
  Fellow3_VehicleLights : Subsystem
  Fellow4_VehicleLights : Subsystem
  Fellow5_VehicleLights : Subsystem
  Fellow6_VehicleLights : Subsystem
  Fellow7_VehicleLights : Subsystem
  Fellow8_VehicleLights : Subsystem
  Fellow9_VehicleLights : Subsystem
  Out1 : Outport  VectorParamsAs1DForOutWhenUnconnected=off
  wires:
  Bus Creator2/1 -> Out1/1  "FellowVehicleLights"
  Fellow30_VehicleLights/1(Out1) -> Bus Creator2/30  "Fellow30_VehicleLights"
  Fellow29_VehicleLights/1(Out1) -> Bus Creator2/29  "Fellow29_VehicleLights"
  Fellow28_VehicleLights/1(Out1) -> Bus Creator2/28  "Fellow28_VehicleLights"
  Fellow27_VehicleLights/1(Out1) -> Bus Creator2/27  "Fellow27_VehicleLights"
  Fellow26_VehicleLights/1(Out1) -> Bus Creator2/26  "Fellow26_VehicleLights"
  Fellow25_VehicleLights/1(Out1) -> Bus Creator2/25  "Fellow25_VehicleLights"
  Fellow24_VehicleLights/1(Out1) -> Bus Creator2/24  "Fellow24_VehicleLights"
  Fellow23_VehicleLights/1(Out1) -> Bus Creator2/23  "Fellow23_VehicleLights"
  Fellow22_VehicleLights/1(Out1) -> Bus Creator2/22  "Fellow22_VehicleLights"
  Fellow21_VehicleLights/1(Out1) -> Bus Creator2/21  "Fellow21_VehicleLights"
  Fellow20_VehicleLights/1(Out1) -> Bus Creator2/20  "Fellow20_VehicleLights"
  Fellow19_VehicleLights/1(Out1) -> Bus Creator2/19  "Fellow19_VehicleLights"
  Fellow18_VehicleLights/1(Out1) -> Bus Creator2/18  "Fellow18_VehicleLights"
  Fellow17_VehicleLights/1(Out1) -> Bus Creator2/17  "Fellow17_VehicleLights"
  Fellow16_VehicleLights/1(Out1) -> Bus Creator2/16  "Fellow16_VehicleLights"
  Fellow15_VehicleLights/1(Out1) -> Bus Creator2/15  "Fellow15_VehicleLights"
  Fellow14_VehicleLights/1(Out1) -> Bus Creator2/14  "Fellow14_VehicleLights"
  Fellow13_VehicleLights/1(Out1) -> Bus Creator2/13  "Fellow13_VehicleLights"
  Fellow12_VehicleLights/1(Out1) -> Bus Creator2/12  "Fellow12_VehicleLights"
  Fellow11_VehicleLights/1(Out1) -> Bus Creator2/11  "Fellow11_VehicleLights"
  Fellow10_VehicleLights/1(Out1) -> Bus Creator2/10  "Fellow10_VehicleLights"
  Fellow9_VehicleLights/1(Out1) -> Bus Creator2/9  "Fellow9_VehicleLights"
  Fellow8_VehicleLights/1(Out1) -> Bus Creator2/8  "Fellow8_VehicleLights"
  Fellow7_VehicleLights/1(Out1) -> Bus Creator2/7  "Fellow7_VehicleLights"
  Fellow6_VehicleLights/1(Out1) -> Bus Creator2/6  "Fellow6_VehicleLights"
  Fellow5_VehicleLights/1(Out1) -> Bus Creator2/5  "Fellow5_VehicleLights"
  Fellow4_VehicleLights/1(Out1) -> Bus Creator2/4  "Fellow4_VehicleLights"
  Fellow3_VehicleLights/1(Out1) -> Bus Creator2/3  "Fellow3_VehicleLights"
  Fellow2_VehicleLights/1(Out1) -> Bus Creator2/2  "Fellow2_VehicleLights"
  Fellow1_VehicleLights/1(Out1) -> Bus Creator2/1  "Fellow1_VehicleLights"

== system ASM_Traffic_MultiCore/Environment/Traffic/UserInterface/PAR_Plant/TrafficControl ==
  Sw_TrafficEnable[0Off|1On] : Constant
  Out1 : Outport  VectorParamsAs1DForOutWhenUnconnected=off
  wires:
  Sw_TrafficEnable[0Off|1On]/1 -> Out1/1  "Sw_TrafficEnable[0Off|1On]"

== system ASM_Traffic_MultiCore/Environment/Traffic/UserInterface/PAR_Plant/V2X ==
  Bus Creator : BusCreator  Inputs=1
  Detect Increase : simulink/Logic and Bit Operations/Detect Increase  vinit=0.0  OutDataTypeStr=uint8
  Reset[0|1] : Constant  Value=0  OutDataTypeStr=uint8
  Out1 : Outport  VectorParamsAs1DForOutWhenUnconnected=off
  wires:
  Bus Creator/1 -> Out1/1  "V2X"
  Detect Increase/1 -> Bus Creator/1  "Reset[0|1]"
  Reset[0|1]/1 -> Detect Increase/1  "Reset[0|1]"

== system ASM_Traffic_MultiCore/VehicleDynamics/Control/SoftECU_Brake/Map_Inputs/Maneuver ==
  note: Initial value is set
      | to ESP (2)
  note: Initial value is set
      | to ASR On (1)
  ECU_Commands[] : Inport
  Reset[0|1] : Inport  Port=2
  Add : Sum  Inputs=+++
  Data Type Conversion : DataTypeConversion  SaturateOnIntegerOverflow=off  RndMeth=Floor
  Data Type Conversion1 : DataTypeConversion  SaturateOnIntegerOverflow=off  RndMeth=Floor
  Fcn10 : Fcn  Expr=u(1)==2011
  Fcn2 : Fcn  Expr=u(1)==2010
  Fcn3 : Fcn  Expr=u(1)==2021
  Fcn4 : Fcn  Expr=u(1)==2020
  Fcn9 : Fcn  Expr=u(1)==2012
  Gain : Gain  Gain=0
  Gain1 : Gain
  Gain2 : Gain  Gain=2
  Logical Operator1 : Logic  Operator=OR  AllPortsSameDT=off  OutDataTypeStr=boolean
  Logical Operator2 : Logic  AllPortsSameDT=off  OutDataTypeStr=boolean
  Logical Operator3 : Logic  Operator=NOT  Inputs=1  AllPortsSameDT=off  OutDataTypeStr=boolean
  Logical Operator : Logic  Operator=OR  Inputs=4  AllPortsSameDT=off  OutDataTypeStr=boolean
  Memory : Memory  InitialCondition=2
  S_R_FlipFlop : Subsystem  mask(S_R_FlipFlop){initial_condition=1}
      mask prompts: initial_condition "Initial condition (state of Q):"
      mask help: S-R Flip-Flop Block
  Sw_ESP_Default : Constant  Value=2
  Switch : Switch  Threshold=0.5  SaturateOnIntegerOverflow=off  InputSameDT=off
  Switch1 : Switch  Threshold=0.5  SaturateOnIntegerOverflow=off  InputSameDT=off
  Terminator : Terminator
  pos_edge_detection : Subsystem
  pos_edge_detection1 : Subsystem
  pos_edge_detection2 : Subsystem
  pos_edge_detection3 : Subsystem
  Sw_ESP[0Off|1ABS|2ESP] : Outport  VectorParamsAs1DForOutWhenUnconnected=off
  Sw_ASR0Off|1On] : Outport  Port=2  VectorParamsAs1DForOutWhenUnconnected=off
  wires:
  Fcn3/1 -> Logical Operator2/2
  Logical Operator3/1 -> Logical Operator2/1
  Logical Operator2/1 -> Data Type Conversion1/1
  Data Type Conversion1/1 -> S_R_FlipFlop/2(R)
  Data Type Conversion/1 -> S_R_FlipFlop/1(S)
  ECU_Commands[]/1 -> Fcn3/1, Fcn4/1, Fcn9/1, Fcn10/1, Fcn2/1
  Fcn9/1 -> pos_edge_detection/1(In1), Gain2/1
  Fcn10/1 -> pos_edge_detection1/1(In1), Gain1/1
  Fcn2/1 -> pos_edge_detection2/1(In1), Gain/1
  pos_edge_detection/1(Out1) -> Logical Operator/1
  pos_edge_detection1/1(Out1) -> Logical Operator/2
  pos_edge_detection2/1(Out1) -> Logical Operator/3
  Gain2/1 -> Add/3
  Gain1/1 -> Add/2
  Gain/1 -> Add/1
  Logical Operator/1 -> Switch/2
  Switch/1 -> Sw_ESP[0Off|1ABS|2ESP]/1, Memory/1
  Memory/1 -> Switch/3
  pos_edge_detection3/1(Out1) -> Switch1/2, Logical Operator/4
  Add/1 -> Switch1/3
  Reset[0|1]/1 -> Logical Operator1/1, Logical Operator3/1, pos_edge_detection3/1(In1)
  Switch1/1 -> Switch/1
  Sw_ESP_Default/1 -> Switch1/1
  S_R_FlipFlop/1(Q) -> Sw_ASR0Off|1On]/1
  Fcn4/1 -> Logical Operator1/2
  Logical Operator1/1 -> Data Type Conversion/1
  S_R_FlipFlop/2(!Q) -> Terminator/1

== system ASM_Traffic_MultiCore/VehicleDynamics/Control/SoftECU_Brake/Soft_ECU_Brake/ASMSignalCollector ==
  Bus Creator : BusCreator  Inputs=1
  ASMSignalBus : Outport  VectorParamsAs1DForOutWhenUnconnected=off
  wires:
  Bus Creator/1 -> ASMSignalBus/1  "SoftECU_Brake"
  [ASMBUS_SoftECU_BrakeDesired] -> Bus Creator/1

== system ASM_Traffic_MultiCore/VehicleDynamics/Control/SoftECU_Brake/Soft_ECU_Brake/avoid_incomplete_trace2source ==
  In1 : Inport
  DummyGain : Gain
  Out1 : Outport
  wires:
  DummyGain/1 -> Out1/1
  In1/1 -> DummyGain/1

== system ASM_Traffic_MultiCore/VehicleDynamics/Control/UserInterface/DISP_Control/ECU_Brake ==
  In : Inport
  Bus Selector1 : BusSelector  OutputSignals=SoftECU_Brake.DesiredBrakePressure.Enable_p_Brake_Desired[0|1],SoftECU_Brake.DesiredBrakePressure.p_Brake_Desired[bar]
  Enable_p_Brake_Desired[0|1] : Subsystem
      mask Display: disp('')
  SoftECU_Brake : Scope  NumInputPorts=2
      settings: TimeSpan=5  ActiveDisplayYMinimum=-1  ActiveDisplayYMaximum=1  DataLoggingMaxPoints=20000  DataLoggingDecimation=10  DataLoggingVariableName=ScopeData4  DataLoggingSaveFormat=Array
  p_Brake_Desired[bar] : Subsystem
      mask Display: disp('')
  wires:
  Enable_p_Brake_Desired[0|1]/1(Out1) -> SoftECU_Brake/1  "Enable_p_Brake_Desired[0|1]"
  In/1 -> Bus Selector1/1
  Bus Selector1/1 -> Enable_p_Brake_Desired[0|1]/1(In1)  "<Enable_p_Brake_Desired[0|1]>"
  p_Brake_Desired[bar]/1(Out1) -> SoftECU_Brake/2  "p_Brake_Desired[bar]"
  Bus Selector1/2 -> p_Brake_Desired[bar]/1(In1)  "<p_Brake_Desired[bar]>"

== system ASM_Traffic_MultiCore/VehicleDynamics/Control/UserInterface/PAR_Control/ECU_Brake ==
  Bus Creator : BusCreator  Inputs=1
  SoftECU_ESP_Switches : Subsystem
      mask Display: disp('SoftECU ESP Switches')
  SoftECU_Brake : Outport  VectorParamsAs1DForOutWhenUnconnected=off
  wires:
  Bus Creator/1 -> SoftECU_Brake/1  "SoftECU_Brake"
  SoftECU_ESP_Switches/1(Out1) -> Bus Creator/1
